simulink model "heli_p2_lqri"  (R2020b)
settings: Solver=ode1  StartTime=0.0  StopTime=30  FixedStep=0.002  RelTol=1e-3  EnableMultiTasking=on
PostLoadFcn:
  | qc_set_target_type(getConfigSet(bdroot, 'QUARC Default Target Configuration'));
values from neighbouring files (symbols this model uses):
  edot_pulse = 0.1    [p2_lqr.m]    (also in p2_lqri.m)
  F = [K(1,1) K(1,3) ... (first row only)    [p2_lqr.m]    (also in p2_lqri.m = zeros(2))
  Joystick_gain_x = 1    [init_heli_1_2.m]    (also in init_heli_3_10.m)
  Joystick_gain_y = -1    [init_heli_1_2.m]    (also in init_heli_3_10.m)
  K = lqr(A_lqr, B_lqr, Q, R)    [p2_compare.m]    (also in p2_lqr.m; p2_lqri.m = lqr(A_lqri, B_lqri, Q, R); p2_report_figs.m = lqr(A, B, Q, R); p2_report_figs_backup.m = lqr(A, B, Q, R))
  pc_step = 0.3    [p2_lqr.m]    (also in p2_lqri.m)
  pulse_len = 3    [p2_lqr.m]    (also in p2_lqri.m)
  Vd_trim = 0    [heli_params.m]
  Vs0 = 7.3    [Task_2.m]    (also in heli_params.m)
undefined symbols (not defined in the file or in its folder): HIL, qc_get_step_size
libraries: quarc_library x4
settings Model: SimulationMode=external  ExtModeTrigDuration=50000  Creator=Rchan  LastModifiedBy=thorof
settings SolverCC: PositivePriorityOrder=on
settings DataIOCC: LimitDataPoints=on  SaveFormat=Array  SignalLoggingSaveFormat=ModelDataLogs  ReturnWorkspaceOutputs=off
settings OptimizationCC: ExpressionDepthLimit=2147483647  InitFltsAndDblsToZero=on  LifeSpan=inf
settings DebuggingCC: SaveWithParameterizedLinksMsg=none  UnderspecifiedInitializationDetection=Classic  MergeDetectMultiDrivingBlocksExec=none  SolverPrmCheckMsg=warning  MultiTaskDSMMsg=warning  MultiTaskCondExecSysMsg=none  FcnCallInpInsideContextMsg=warning  AllowSymbolicDim=off  StateNameClashWarn=warning  SFUnexpectedBacktrackingDiag=warning  SFNoUnconditionalDefaultTransitionDiag=warning  SFExecutionAtInitializationDiag=none  ArithmeticOperatorsInVariantConditions=warning
settings HardwareCC: ProdBitPerPointer=32  ProdBitPerSizeT=32  ProdBitPerPtrDiffT=32  ProdLargestAtomicFloat=None  ProdIntDivRoundTo=Undefined  ProdEndianess=Unspecified  ProdWordSize=32  ProdHWDeviceType=32-bit Generic
settings ModelReferenceCC: PropagateSignalLabelsOutOfModel=off
settings SFSimCC: SimUseLocalCustomCode=off  CustomCodeUndefinedFunction=UseInterfaceOnly
settings RTWCC: Description=QUARC Win64 Target  SystemTargetFile=quarc_win64.tlc  TemplateMakefile=quarc_default_tmf  RTWUseLocalCustomCode=off
settings CodeAppCC: StateflowObjectComments=on
settings GRTTargetCC: TargetLangStandard=C89/C90 (ANSI)  ParMdlRefBuildCompliant=off  CompOptLevelCompliant=off  CombineOutputUpdateFcns=off  MatFileLogging=off  GRTInterface=on  UseToolchainInfoCompliant=off  ExtMode=on  ExtModeMexFile=quarc_comm
settings ConfigComp: CovMetricSettings=dw  CovSaveCumulativeToWorkspaceVar=on  CovSaveSingleToWorkspaceVar=on  CovExternalEMLEnable=off  CovSFcnEnable=off

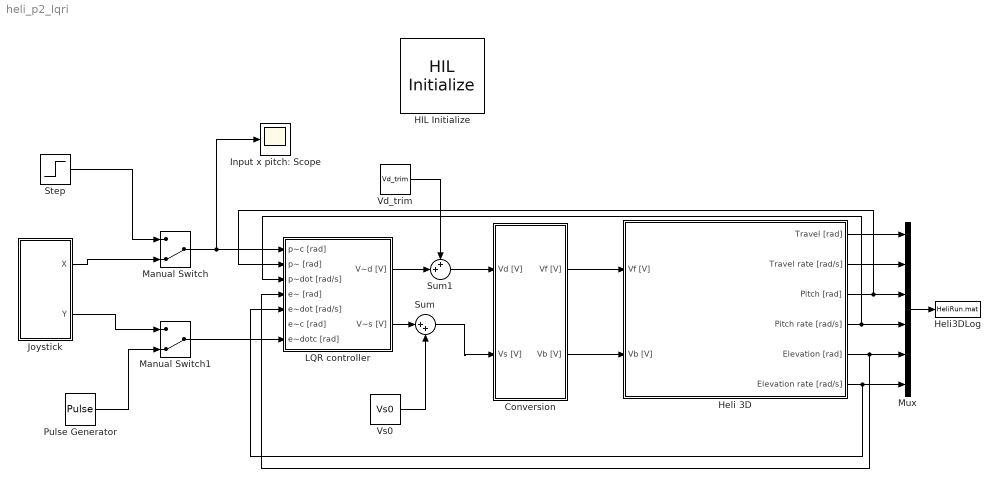
== system heli_p2_lqri ==
  Conversion : Subsystem
  HIL Initialize : quarc_library/Data Acquisition/Generic/Configuration/HIL Initialize  Priority=-99  object_name=HIL-1  board_type=q8_usb  board_number=0  board_options=update_rate=normal;decimation=1  exclusive=off  active=off  hardware_clocks=[0:2]  clock_modes=[]  initial_clock_frequencies=[]  set_clock_params_at_start=off  set_clock_params_at_switch_in=off  set_clock_frequencies_at_start=off  set_clock_frequencies_at_switch_in=off  analog_input_channels=[0:7]  analog_input_configurations=[]  analog_input_maximums=10  analog_input_minimums=-10  set_analog_input_params_at_start=on  set_analog_input_params_at_switch_in=off  analog_output_channels=[0:7]  analog_output_maximums=10  analog_output_minimums=-10  initial_analog_outputs=[0]  final_analog_outputs=[0]  watchdog_analog_outputs=0  set_analog_output_params_at_start=on  set_analog_output_params_at_switch_in=off  set_analog_outputs_at_start=on  set_analog_outputs_at_switch_in=off  set_analog_outputs_at_terminate=on  set_analog_outputs_at_switch_out=off  set_analog_outputs_on_watchdog=off  digital_input_channels=[]  digital_output_channels=[]  digital_output_configuration=[]  initial_digital_outputs=[1]  final_digital_outputs=[1]  watchdog_digital_outputs=[1]  set_digital_output_params_at_start=off  set_digital_output_params_at_switch_in=off  set_digital_outputs_at_start=on  set_digital_outputs_at_switch_in=off  set_digital_outputs_at_terminate=on  set_digital_outputs_at_switch_out=off  set_digital_outputs_on_watchdog=off  encoder_channels=[0:7]  quadrature=[4]  encoder_filter_frequency=[]  initial_encoder_counts=[0]  set_encoder_params_at_start=on  set_encoder_params_at_switch_in=off  set_encoder_counts_at_start=on  set_encoder_counts_at_switch_in=off  pwm_channels=[0:7]  pwm_modes=0  pwm_frequency=99.532799999999995e6/4095  pwm_configuration=[0]  pwm_alignment=[0]  pwm_polarity=[1]  pwm_leading_deadband=[0]  pwm_trailing_deadband=[0]  initial_pwm_outputs=[0]  final_pwm_outputs=[0]  watchdog_pwm_outputs=[0]  set_pwm_params_at_start=on  set_pwm_params_at_switch_in=off  set_pwm_outputs_at_start=on  set_pwm_outputs_at_switch_in=off  set_pwm_outputs_at_terminate=on  set_pwm_outputs_at_switch_out=off  set_pwm_outputs_on_watchdog=off  other_output_channels=[]  initial_other_outputs=[]  final_other_outputs=[]  watchdog_other_outputs=[]  set_other_outputs_at_start=off  set_other_outputs_at_switch_in=off  set_other_outputs_at_terminate=off  set_other_outputs_at_switch_out=off  set_other_outputs_on_watchdog=off
  Heli 3D : Subsystem
  Heli3DLog : ToFile  Filename=HeliRun.mat
  Input x pitch: Scope : Scope
  Joystick : Subsystem
  LQR controller : Subsystem
  Manual Switch : ManualSwitch  CurrentSetting=0
  Manual Switch1 : ManualSwitch  CurrentSetting=0
  Mux : Mux  Inputs=6
  Pulse Generator : DiscretePulseGenerator  PulseType=Time based  Amplitude=edot_pulse  Period=20  PulseWidth=pulse_len/20*100  PhaseDelay=5
  Step : Step  Time=5  After=pc_step  SampleTime=0
  Sum : Sum  Inputs=|++
  Sum1 : Sum  Inputs=++|
  Vd_trim : Constant  Value=Vd_trim
  Vs0 : Constant  Value=Vs0
  wires:
  Conversion/2(Vb [V]) -> Heli 3D/2(Vb [V])
  Conversion/1(Vf [V]) -> Heli 3D/1(Vf [V])
  Heli 3D/1(Travel [rad]) -> Mux/1
  Heli 3D/2(Travel rate [rad/s]) -> Mux/2
  Heli 3D/3(Pitch [rad]) -> LQR controller/2(p~ [rad]), Mux/3
  Heli 3D/4(Pitch rate [rad/s]) -> LQR controller/3(p~dot [rad/s]), Mux/4
  Heli 3D/5(Elevation [rad]) -> LQR controller/4(e~ [rad]), Mux/5
  Heli 3D/6(Elevation rate [rad/s]) -> LQR controller/5(e~dot [rad/s]), Mux/6
  Mux/1 -> Heli3DLog/1
  Sum/1 -> Conversion/2(Vs [V])
  Step/1 -> Manual Switch/1
  LQR controller/2(V~s [V]) -> Sum/1
  Vs0/1 -> Sum/2
  LQR controller/1(V~d [V]) -> Sum1/2
  Sum1/1 -> Conversion/1(Vd [V])
  Vd_trim/1 -> Sum1/1
  Joystick/1(X) -> Manual Switch/2
  Joystick/2(Y) -> Manual Switch1/1
  Manual Switch1/1 -> LQR controller/7(e~dotc [rad])
  Pulse Generator/1 -> Manual Switch1/2
  Manual Switch/1 -> Input x pitch: Scope/1, LQR controller/1(p~c [rad])

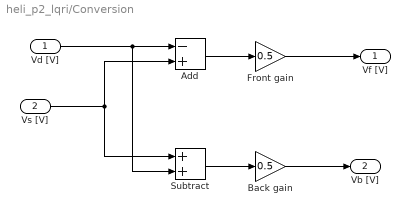
== system heli_p2_lqri/Conversion ==
  Vd [V] : Inport
  Vs [V] : Inport  Port=2
  Add : Sum  Inputs=-+
  Back gain : Gain  Gain=0.5
  Front gain : Gain  Gain=0.5
  Subtract : Sum
  Vf [V] : Outport
  Vb [V] : Outport  Port=2
  wires:
  Vd [V]/1 -> Subtract/2, Add/1
  Vs [V]/1 -> Subtract/1, Add/2
  Subtract/1 -> Back gain/1
  Back gain/1 -> Vb [V]/1
  Add/1 -> Front gain/1
  Front gain/1 -> Vf [V]/1

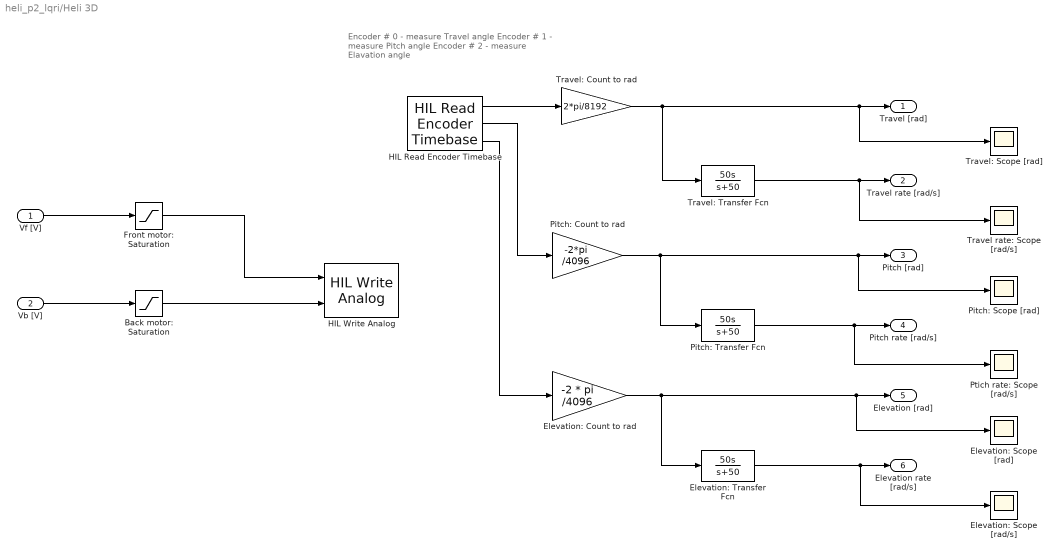
== system heli_p2_lqri/Heli 3D ==
  note: Encoder # 0 - measure Travel angle
      | Encoder # 1 - measure Pitch angle
      | Encoder # 2 - measure Elavation angle
  Vf [V] : Inport
  Vb [V] : Inport  Port=2
  Back motor: Saturation : Saturate  UpperLimit=5  LowerLimit=-5
  Elevation: Count to rad : Gain  Gain=-2 * pi /4096
  Elevation: Scope [rad/s] : Scope
  Elevation: Scope [rad] : Scope
  Elevation: Transfer Fcn : TransferFcn  Numerator=[50 0]  Denominator=[1 50]
  Front motor: Saturation : Saturate  UpperLimit=5  LowerLimit=-5
  HIL Read Encoder Timebase : quarc_library/Data Acquisition/Generic/Timebases/HIL Read Encoder Timebase  object_name=HIL-1  clock=0  channels=[0:2]  active=on  vector_output=off  data_type_mode=Inherit via back propagation  data_type=double  overflow_mode=Error on overflow  samples_in_buffer=max(ceil(1/qc_get_step_size), 1)
  HIL Write Analog : quarc_library/Data Acquisition/Generic/Immediate I//O/HIL Write Analog  object_name=HIL-1  channels=[0:1]  sample_time=-1  active=off  vector_input=off
  Pitch: Count to rad : Gain  Gain=-2*pi /4096
  Pitch: Scope [rad] : Scope
  Pitch: Transfer Fcn : TransferFcn  Numerator=[50 0]  Denominator=[1 50]
  Ptich rate: Scope [rad/s] : Scope
  Travel rate: Scope [rad/s] : Scope
  Travel: Count to rad : Gain  Gain=2*pi/8192
  Travel: Scope [rad] : Scope
  Travel: Transfer Fcn : TransferFcn  Numerator=[50 0]  Denominator=[1 50]
  Travel [rad] : Outport
  Travel rate [rad/s] : Outport  Port=2
  Pitch [rad] : Outport  Port=3
  Pitch rate [rad/s] : Outport  Port=4
  Elevation [rad] : Outport  Port=5
  Elevation rate [rad/s] : Outport  Port=6
  wires:
  HIL Read Encoder Timebase/1 -> Travel: Count to rad/1
  HIL Read Encoder Timebase/2 -> Pitch: Count to rad/1
  HIL Read Encoder Timebase/3 -> Elevation: Count to rad/1
  Travel: Count to rad/1 -> Travel: Scope [rad]/1, Travel [rad]/1, Travel: Transfer Fcn/1
  Travel: Transfer Fcn/1 -> Travel rate: Scope [rad/s]/1, Travel rate [rad/s]/1
  Pitch: Count to rad/1 -> Pitch: Transfer Fcn/1, Pitch: Scope [rad]/1, Pitch [rad]/1
  Pitch: Transfer Fcn/1 -> Ptich rate: Scope [rad/s]/1, Pitch rate [rad/s]/1
  Elevation: Count to rad/1 -> Elevation: Transfer Fcn/1, Elevation: Scope [rad]/1, Elevation [rad]/1
  Elevation: Transfer Fcn/1 -> Elevation: Scope [rad/s]/1, Elevation rate [rad/s]/1
  Vf [V]/1 -> Front motor: Saturation/1
  Vb [V]/1 -> Back motor: Saturation/1
  Front motor: Saturation/1 -> HIL Write Analog/1
  Back motor: Saturation/1 -> HIL Write Analog/2

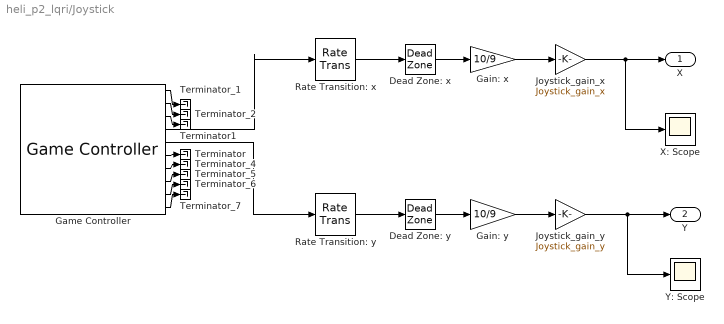
== system heli_p2_lqri/Joystick ==
  Dead Zone: x : DeadZone  LowerValue=-0.1  UpperValue=0.1  SaturateOnIntegerOverflow=on
  Dead Zone: y : DeadZone  LowerValue=-0.1  UpperValue=0.1  SaturateOnIntegerOverflow=on
  Gain: x : Gain  Gain=10/9
  Gain: y : Gain  Gain=10/9
  Game Controller : quarc_library/Devices/Peripherals/Target/Game Controller  controller=1  buffer_size=12  deadzone=[]  saturation=[]  sample_time=max(qc_get_step_size, 0.01)  auto_center=off  enabled=on
      settings: SourceProductName=QUARC Targets
  Joystick_gain_x : Gain  Gain=Joystick_gain_x
  Joystick_gain_y : Gain  Gain=Joystick_gain_y
  Rate Transition: x : RateTransition
  Rate Transition: y : RateTransition
  Terminator : Terminator
  Terminator1 : Terminator
  Terminator_{1..2,4..7} (6 alike) : Terminator
  X: Scope : Scope
  Y: Scope : Scope
  X : Outport
  Y : Outport  Port=2
  wires:
  Rate Transition: y/1 -> Dead Zone: y/1
  Rate Transition: x/1 -> Dead Zone: x/1
  Game Controller/5 -> Rate Transition: y/1
  Game Controller/4 -> Rate Transition: x/1
  Game Controller/1 -> Terminator_1/1
  Game Controller/2 -> Terminator_2/1
  Game Controller/7 -> Terminator_4/1
  Game Controller/8 -> Terminator_5/1
  Game Controller/9 -> Terminator_6/1
  Game Controller/10 -> Terminator_7/1
  Game Controller/3 -> Terminator1/1
  Game Controller/6 -> Terminator/1
  Dead Zone: x/1 -> Gain: x/1
  Dead Zone: y/1 -> Gain: y/1
  Gain: x/1 -> Joystick_gain_x/1
  Gain: y/1 -> Joystick_gain_y/1
  Joystick_gain_x/1 -> X/1, X: Scope/1
  Joystick_gain_y/1 -> Y: Scope/1, Y/1

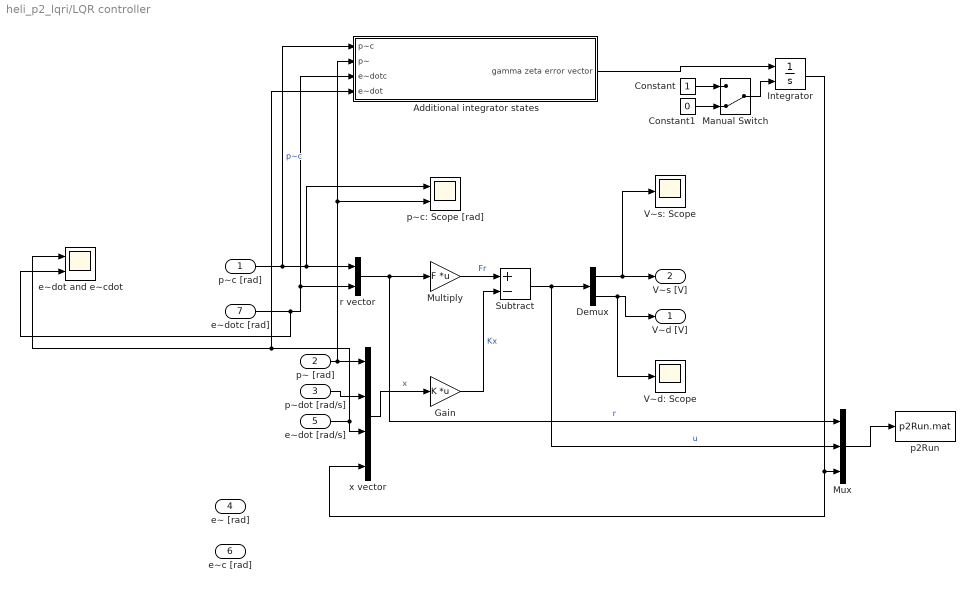
== system heli_p2_lqri/LQR controller ==
  p~c [rad] : Inport
  p~ [rad] : Inport  Port=2
  p~dot [rad/s] : Inport  Port=3
  e~ [rad] : Inport  Port=4
  e~dot [rad/s] : Inport  Port=5
  e~c [rad] : Inport  Port=6
  e~dotc [rad] : Inport  Port=7
  Additional integrator states : Subsystem
  Constant : Constant
  Constant1 : Constant  Value=0
  Demux : Demux  Outputs=2
  Gain : Gain  Gain=K  Multiplication=Matrix(K*u)
  Integrator : Integrator  ExternalReset=level
  Manual Switch : ManualSwitch  CurrentSetting=0
  Multiply : Gain  Gain=F  Multiplication=Matrix(K*u)
  Mux : Mux  Inputs=3
  Subtract : Sum  Inputs=+-
  V~d: Scope : Scope
  V~s: Scope : Scope
  e~dot and e~cdot : Scope  NumInputPorts=2
  p2Run : ToFile  Filename=p2Run.mat
  p~c: Scope [rad] : Scope  NumInputPorts=2
  r vector : Mux  Inputs=2
  x vector : Mux
  V~d [V] : Outport  InitialOutput=0
  V~s [V] : Outport  Port=2  InitialOutput=0
  wires:
  p~c [rad]/1 -> Additional integrator states/1(p~c), p~c: Scope [rad]/1, r vector/1  "p~c"
  e~dotc [rad]/1 -> e~dot and e~cdot/2, r vector/2, Additional integrator states/3(e~dotc)
  r vector/1 -> Mux/1, Multiply/1  "r"
  Multiply/1 -> Subtract/1  "Fr"
  x vector/1 -> Gain/1  "x"
  Gain/1 -> Subtract/2  "Kx"
  e~dot [rad/s]/1 -> Additional integrator states/4(e~dot), e~dot and e~cdot/1, x vector/3
  p~ [rad]/1 -> Additional integrator states/2(p~), p~c: Scope [rad]/2, x vector/1
  p~dot [rad/s]/1 -> x vector/2
  Subtract/1 -> Mux/2, Demux/1  "u"
  Demux/1 -> V~s: Scope/1, V~s [V]/1
  Demux/2 -> V~d: Scope/1, V~d [V]/1
  Mux/1 -> p2Run/1
  Additional integrator states/1(gamma zeta error vector) -> Integrator/1
  Integrator/1 -> Mux/3, x vector/4
  Manual Switch/1 -> Integrator/2
  Constant/1 -> Manual Switch/1
  Constant1/1 -> Manual Switch/2

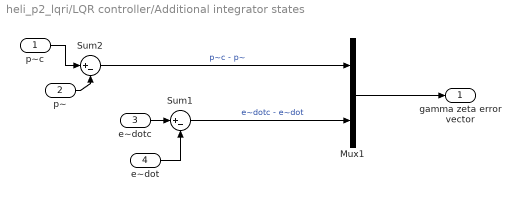
== system heli_p2_lqri/LQR controller/Additional integrator states ==
  p~c : Inport
  p~ : Inport  Port=2
  e~dotc : Inport  Port=3
  e~dot : Inport  Port=4
  Mux1 : Mux  Inputs=2
  Sum1 : Sum  Inputs=|+-
  Sum2 : Sum  Inputs=|+-
  gamma zeta error vector : Outport
  wires:
  p~c/1 -> Sum2/1
  Sum2/1 -> Mux1/1  "p~c - p~"
  p~/1 -> Sum2/2
  Mux1/1 -> gamma zeta error vector/1
  Sum1/1 -> Mux1/2  "e~dotc - e~dot"
  e~dotc/1 -> Sum1/1
  e~dot/1 -> Sum1/2
